simulink model "heli_q8_R_matrix_measurments"  (R2020b)
settings: Solver=ode1  StartTime=0.0  StopTime=inf  FixedStep=0.002  RelTol=1e-3  EnableMultiTasking=on
PostLoadFcn:
  | qc_set_target_type(getConfigSet(bdroot, 'QUARC Default Target Configuration'));
values from neighbouring files (symbols this model uses):
  A_obs = [0 1 0 0 0 ... (first row only)    [init_heli_R_matrix_measurments.m]
  B_obs = [0 0 ... (first row only)    [init_heli_R_matrix_measurments.m]
  C = [1 0 0 0 0 ... (first row only)    [init_heli_R_matrix_measurments.m]
  elevation_offset = 0.5    [init_heli.m]    (also in init_heli_R_matrix_measurments.m)
  F = [K(1,1) K(1,3) ... (first row only)    [init_heli.m]    (also in init_heli_R_matrix_measurments.m)
  Joystick_gain_x = 2    [init_heli.m]    (also in init_heli_R_matrix_measurments.m)
  Joystick_gain_y = -0.5    [init_heli.m]    (also in init_heli_R_matrix_measurments.m)
  K = lqr(A, B, Q, R)    [init_heli.m]    (also in init_heli_R_matrix_measurments.m)
  L = place(A_obs', C', p)'    [init_heli_R_matrix_measurments.m]
undefined symbols (not defined in the file or in its folder): HIL, qc_get_step_size
libraries: quarc_library x9, simulink x4, cstblocks x2, pid_lib x1
settings Model: SimulationMode=external  ExtModeTrigDuration=600000  Creator=Rchan  LastModifiedBy=wiktorjr
settings SolverCC: PositivePriorityOrder=on
settings DataIOCC: LimitDataPoints=on  SaveFormat=Array  SignalLoggingSaveFormat=ModelDataLogs  ReturnWorkspaceOutputs=off
settings OptimizationCC: ExpressionDepthLimit=2147483647  InitFltsAndDblsToZero=on  LifeSpan=inf
settings DebuggingCC: SaveWithParameterizedLinksMsg=none  UnderspecifiedInitializationDetection=Classic  MergeDetectMultiDrivingBlocksExec=none  SolverPrmCheckMsg=warning  MultiTaskDSMMsg=warning  MultiTaskCondExecSysMsg=none  FcnCallInpInsideContextMsg=warning  AllowSymbolicDim=off  StateNameClashWarn=warning  SFUnexpectedBacktrackingDiag=warning  SFNoUnconditionalDefaultTransitionDiag=warning  SFExecutionAtInitializationDiag=none  ArithmeticOperatorsInVariantConditions=warning
settings HardwareCC: ProdBitPerPointer=32  ProdBitPerSizeT=32  ProdBitPerPtrDiffT=32  ProdLargestAtomicFloat=None  ProdIntDivRoundTo=Undefined  ProdEndianess=Unspecified  ProdWordSize=32  ProdHWDeviceType=32-bit Generic
settings ModelReferenceCC: PropagateSignalLabelsOutOfModel=off
settings SFSimCC: SimUseLocalCustomCode=off  CustomCodeUndefinedFunction=UseInterfaceOnly
settings RTWCC: Description=QUARC Win64 Target  SystemTargetFile=quarc_win64.tlc  TemplateMakefile=quarc_default_tmf  RTWUseLocalCustomCode=off
settings CodeAppCC: StateflowObjectComments=on
settings GRTTargetCC: TargetLangStandard=C89/C90 (ANSI)  ParMdlRefBuildCompliant=off  CompOptLevelCompliant=off  CombineOutputUpdateFcns=off  MatFileLogging=off  GRTInterface=on  UseToolchainInfoCompliant=off  ExtMode=on  ExtModeMexFile=quarc_comm
settings ConfigComp: CovMetricSettings=dw  CovSaveCumulativeToWorkspaceVar=on  CovSaveSingleToWorkspaceVar=on  CovExternalEMLEnable=off  CovSFcnEnable=off

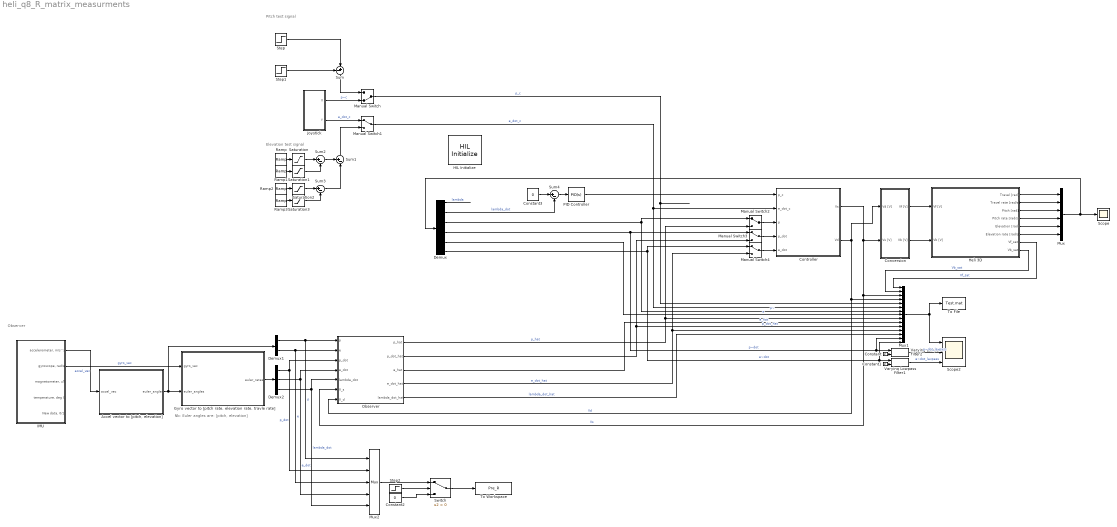
== system heli_q8_R_matrix_measurments ==
  note: Observer
  note: Pitch test signal
  note: Elevation test signal
  note: Nb: Euler angles are: [pitch, elevation]
  "Accel vector to [pitch, elevation]" : MATLAB Function  TreatAsAtomicUnit=on
  Constant : Constant  Value=2
  Constant1 : Constant  Value=2
  Constant2 : Constant  Value=0
  Constant3 : Constant  Value=0
  Controller : Subsystem
  Conversion : Subsystem
  Demux : Demux  Outputs=6
  Demux1 : Demux  Outputs=2
  Demux2 : Demux  Outputs=3
  "Gyro vector to [pitch rate, elevation rate, travle rate]" : MATLAB Function  TreatAsAtomicUnit=on
  HIL Initialize : quarc_library/Data Acquisition/Generic/Configuration/HIL Initialize  Priority=-99  object_name=HIL-1  board_type=q8_usb  board_number=0  board_options=update_rate=normal;decimation=1  exclusive=off  active=off  hardware_clocks=[0:2]  clock_modes=[]  initial_clock_frequencies=[]  set_clock_params_at_start=off  set_clock_params_at_switch_in=off  set_clock_frequencies_at_start=off  set_clock_frequencies_at_switch_in=off  analog_input_channels=[0:7]  analog_input_configurations=[]  analog_input_maximums=10  analog_input_minimums=-10  set_analog_input_params_at_start=on  set_analog_input_params_at_switch_in=off  analog_output_channels=[0:7]  analog_output_maximums=10  analog_output_minimums=-10  initial_analog_outputs=[0]  final_analog_outputs=[0]  watchdog_analog_outputs=0  set_analog_output_params_at_start=on  set_analog_output_params_at_switch_in=off  set_analog_outputs_at_start=on  set_analog_outputs_at_switch_in=off  set_analog_outputs_at_terminate=on  set_analog_outputs_at_switch_out=off  set_analog_outputs_on_watchdog=off  digital_input_channels=[]  digital_output_channels=[]  digital_output_configuration=[]  initial_digital_outputs=[1]  final_digital_outputs=[1]  watchdog_digital_outputs=[1]  set_digital_output_params_at_start=off  set_digital_output_params_at_switch_in=off  set_digital_outputs_at_start=on  set_digital_outputs_at_switch_in=off  set_digital_outputs_at_terminate=on  set_digital_outputs_at_switch_out=off  set_digital_outputs_on_watchdog=off  encoder_channels=[0:7]  quadrature=[4]  encoder_filter_frequency=[]  initial_encoder_counts=[0]  set_encoder_params_at_start=on  set_encoder_params_at_switch_in=off  set_encoder_counts_at_start=on  set_encoder_counts_at_switch_in=off  pwm_channels=[0:7]  pwm_modes=0  pwm_frequency=99.532799999999995e6/4095  pwm_configuration=[0]  pwm_alignment=[0]  pwm_polarity=[1]  pwm_leading_deadband=[0]  pwm_trailing_deadband=[0]  initial_pwm_outputs=[0]  final_pwm_outputs=[0]  watchdog_pwm_outputs=[0]  set_pwm_params_at_start=on  set_pwm_params_at_switch_in=off  set_pwm_outputs_at_start=on  set_pwm_outputs_at_switch_in=off  set_pwm_outputs_at_terminate=on  set_pwm_outputs_at_switch_out=off  set_pwm_outputs_on_watchdog=off  other_output_channels=[]  initial_other_outputs=[]  final_other_outputs=[]  watchdog_other_outputs=[]  set_other_outputs_at_start=off  set_other_outputs_at_switch_in=off  set_other_outputs_at_terminate=off  set_other_outputs_at_switch_out=off  set_other_outputs_on_watchdog=off
  Heli 3D : Subsystem
  IMU : Subsystem
  Joystick : Subsystem
  Manual Switch : ManualSwitch  CurrentSetting=0
  Manual Switch{1..4} (4 alike) : ManualSwitch
  Mux : Mux  Inputs=6
  Mux1 : Mux  Inputs=15
  Mux2 : Mux  Inputs=5
  Observer : Subsystem
  PID Controller : pid_lib/PID Controller  Controller=PID  Form=Parallel  TimeDomain=Continuous-time  UseExternalTs=off  SampleTime=-1  IntegratorMethod=Forward Euler  FilterMethod=Forward Euler  ControllerParametersSource=internal  P=1  I=0.2  D=0  UseFilter=on  N=100  TunerSelectOption=Transfer Function Based (PID Tuner App)  InitialConditionSource=internal  InitialConditionForIntegrator=0  InitialConditionForFilter=0  DifferentiatorICPrevScaledInput=0  ExternalReset=none  TrackingMode=off  Kt=1  LimitOutput=off  SatLimitsSource=internal  UpperSaturationLimit=inf  LowerSaturationLimit=-inf  LinearizeAsGain=on  AntiWindupMode=none  Kb=1  POutMin=[]  POutMax=[]  IOutMin=[]  IOutMax=[]  DOutMin=[]  DOutMax=[]  NOutMin=[]  NOutMax=[]  SumOutMin=[]  SumOutMax=[]  SaturationOutMin=[]  SaturationOutMax=[]  PParamMin=[]  PParamMax=[]  IParamMin=[]  IParamMax=[]  DParamMin=[]  DParamMax=[]  NParamMin=[]  NParamMax=[]  KbParamMin=[]  KbParamMax=[]  KtParamMin=[]  KtParamMax=[]  KbOutMin=[]  KbOutMax=[]  KtOutMin=[]  KtOutMax=[]  IntegratorOutMin=[]  IntegratorOutMax=[]  FilterOutMin=[]  FilterOutMax=[]  SumI1OutMin=[]  SumI1OutMax=[]  SumI2OutMin=[]  SumI2OutMax=[]  SumI3OutMin=[]  SumI3OutMax=[]  SumI4OutMin=[]  SumI4OutMax=[]  SumDOutMin=[]  SumDOutMax=[]  DifferentiatorOutMin=[]  DifferentiatorOutMax=[]  FilterDiffOutCoefMin=[]  FilterDiffOutCoefMax=[]  ReciprocalOutMin=[]  ReciprocalOutMax=[]  SumDenOutMin=[]  SumDenOutMax=[]  SumNumOutMin=[]  SumNumOutMax=[]  DivideOutMin=[]  DivideOutMax=[]  UdiffTsProdOutMin=[]  UdiffTsProdOutMax=[]  NTsProdOutMin=[]  NTsProdOutMax=[]  UintegralTsProdOutMin=[]  UintegralTsProdOutMax=[]  UngainTsProdOutMin=[]  UngainTsProdOutMax=[]  IntegratorContinuousStateAttributes=''  IntegratorStateMustResolveToSignalObject=off  IntegratorRTWStateStorageClass=Auto  FilterContinuousStateAttributes=''  FilterStateMustResolveToSignalObject=off  FilterRTWStateStorageClass=Auto  ParallelPVariant=InternalParameters  IdealPVariant=Disabled  IVariant=InternalParameters  DVariant=InternalParameters  IntegratorVariant=Continuous  SatVariant=Disabled  AWVariant=Passthrough  PCopyVariant=Disabled  TRVariant=Disabled  FdbkBlocksVariant=Forward  IdealPFdbkVariant=Disabled  SatFdbkVariant=Disabled  DerivativeFilterVariant=ContFilter  NVariant=InternalParameters  NCopyVariant=Disabled  FilterICVariant=InternalICsFilter  IntegratorICVariant=InternalICs  ExternalResetVariant=Disabled  TRSumVariant=Passthrough  SumFdbkVariant=Disabled  SumVariant=Sum_PID  TsampFilterVariant=InternalTs  TsampNgainVariant=Passthrough  TsampIntegralVariant=Passthrough  ExternalSaturationOutDataTypeStr=Inherit: Same as second input
  Ramp : simulink/Sources/Ramp  slope=0.03  start=0  InitialOutput=0
  Ramp1 : simulink/Sources/Ramp  slope=0.03  start=4.85  InitialOutput=0
  Ramp2 : simulink/Sources/Ramp  slope=0.03  start=65  InitialOutput=0
  Ramp3 : simulink/Sources/Ramp  slope=0.03  start=70  InitialOutput=0
  Saturation : Saturate  UpperLimit=0.15  LowerLimit=0
  Saturation1 : Saturate  UpperLimit=0.15  LowerLimit=0
  Saturation2 : Saturate  UpperLimit=0.15  LowerLimit=0
  Saturation3 : Saturate  UpperLimit=0.13  LowerLimit=0
  Scope : Scope
  Scope2 : Scope  NumInputPorts=3
  Step : Step  Time=10  After=pi/8  SampleTime=0
  Step1 : Step  Time=40  After=pi/8  SampleTime=0
  Step2 : Step  Time=11  SampleTime=0
  Sum : Sum  Inputs=-+|
  Sum1 : Sum  Inputs=+-|
  Sum2 : Sum  Inputs=|+-
  Sum3 : Sum  Inputs=|+-
  Sum4 : Sum  Inputs=|+-
  Switch : Switch  Criteria=u2 > Threshold
  To File : ToFile  Filename=Test.mat
  To Workspace : ToWorkspace  VariableName=Pre_R  SampleTime=-1
  Varying Lowpass Filter1 : cstblocks/Linear Parameter Varying/Varying Lowpass Filter  N=1
  Varying Lowpass Filter2 : cstblocks/Linear Parameter Varying/Varying Lowpass Filter  N=1
  wires:
  Conversion/2(Vb [V]) -> Heli 3D/2(Vb [V])
  Conversion/1(Vf [V]) -> Heli 3D/1(Vf [V])
  Heli 3D/1(Travel [rad]) -> Mux/1
  Heli 3D/2(Travel rate [rad/s]) -> Mux/2
  Heli 3D/3(Pitch [rad]) -> Mux/3
  Heli 3D/4(Pitch rate [rad/s]) -> Mux/4
  Heli 3D/5(Elevation [rad]) -> Mux/5
  Heli 3D/6(Elevation rate [rad/s]) -> Mux/6
  Mux/1 -> Demux/1, Scope/1
  Mux1/1 -> To File/1, Scope2/1
  Controller/2(Vd) -> Conversion/1(Vd [V]), Observer/7(V_d), Mux1/4  "Vd"
  Demux/3 -> Mux1/7, Manual Switch2/1  "p~"
  Demux/4 -> Mux1/14, Varying Lowpass Filter2/1, Manual Switch3/1  "p~dot"
  Demux/6 -> Mux1/15, Varying Lowpass Filter1/1, Manual Switch4/1  "e~dot"
  Manual Switch/1 -> Mux1/5  "p_c"
  Manual Switch1/1 -> Controller/2(e_dot_c), Mux1/6  "e_dot_c"
  Joystick/2(Y) -> Manual Switch1/1  "e_dot_c"
  Joystick/1(X) -> Manual Switch/2  "p~c"
  Controller/1(Vs) -> Conversion/2(Vs [V]), Observer/6(V_s), Mux1/3  "Vs"
  Constant1/1 -> Varying Lowpass Filter1/2
  Constant/1 -> Varying Lowpass Filter2/2
  Varying Lowpass Filter2/1 -> Scope2/2  "p~dot_lavpass"
  Varying Lowpass Filter1/1 -> Scope2/3  "e~dot_lavpass"
  Sum/1 -> Manual Switch/1
  Step/1 -> Sum/2
  Step1/1 -> Sum/1
  Sum1/1 -> Manual Switch1/2
  Ramp/1 -> Saturation/1
  Saturation/1 -> Sum2/1
  Sum2/1 -> Sum1/1
  Ramp1/1 -> Saturation1/1
  Saturation1/1 -> Sum2/2
  Saturation3/1 -> Sum3/2
  Ramp3/1 -> Saturation3/1
  Saturation2/1 -> Sum3/1
  Ramp2/1 -> Saturation2/1
  Sum3/1 -> Sum1/2
  Heli 3D/8(Vb_sat) -> Mux1/2  "Vb_sat"
  Heli 3D/7(Vf_sat) -> Mux1/1  "Vf_sat"
  IMU/1("accelerometer, m/s^2") -> "Accel vector to [pitch, elevation]"/1(accel_vec)  "accel_vec"
  IMU/2("gyroscope, rad/s") -> "Gyro vector to [pitch rate, elevation rate, travle rate]"/1(gyro_vec)  "gyro_vec"
  "Accel vector to [pitch, elevation]"/1(euler_angles) -> Demux1/1, "Gyro vector to [pitch rate, elevation rate, travle rate]"/2(euler_angles)
  "Gyro vector to [pitch rate, elevation rate, travle rate]"/1(euler_rates) -> Demux2/1
  Demux1/1 -> Mux2/1, Observer/1(p)  "p"
  Demux1/2 -> Mux2/3, Observer/2(e)  "e"
  Demux2/1 -> Mux2/2, Observer/3(p_dot)  "p_dot"
  Demux2/2 -> Observer/4(e_dot), Mux2/4  "e_dot"
  Demux2/3 -> Mux2/5, Observer/5(lambda_dot)  "lambda_dot"
  Observer/1(p_hat) -> Manual Switch2/2, Mux1/9  "p_hat"
  Observer/3(e_hat) -> Mux1/10  "e_hat"
  Observer/2(p_dot_hat) -> Manual Switch3/2, Mux1/11  "p_dot_hat"
  Observer/4(e_dot_hat) -> Manual Switch4/2, Mux1/12  "e_dot_hat"
  Observer/5(lambda_dot_hat) -> Mux1/13  "lambda_dot_hat"
  Demux/5 -> Mux1/8  "e"
  Mux2/1 -> Switch/1
  Switch/1 -> To Workspace/1
  Step2/1 -> Switch/2
  Constant2/1 -> Switch/3
  Demux/2 -> Sum4/2  "lambda_dot"
  Demux/1 -> ?  "lambda"
  Manual Switch2/1 -> Controller/3(p)
  Manual Switch3/1 -> Controller/4(p_dot)
  Manual Switch4/1 -> Controller/5(e_dot)
  PID Controller/1 -> Controller/1(p_c)
  Sum4/1 -> PID Controller/1
  Constant3/1 -> Sum4/1

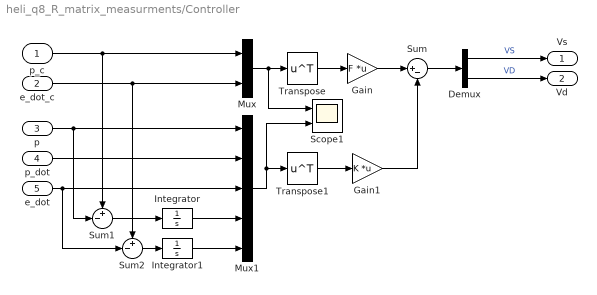
== system heli_q8_R_matrix_measurments/Controller ==
  p_c : Inport
  e_dot_c : Inport  Port=2
  p : Inport  Port=3
  p_dot : Inport  Port=4
  e_dot : Inport  Port=5
  Demux : Demux  Outputs=2
  Gain : Gain  Gain=F  Multiplication=Matrix(K*u) (u vector)
  Gain1 : Gain  Gain=K  Multiplication=Matrix(K*u) (u vector)
  Integrator : Integrator
  Integrator1 : Integrator
  Mux : Mux  Inputs=2
  Mux1 : Mux  Inputs=5
  Scope1 : Scope  NumInputPorts=2
  Sum : Sum  Inputs=|+-
  Sum1 : Sum  Inputs=+-|
  Sum2 : Sum  Inputs=+-|
  Transpose : Math  Operator=transpose  SaturateOnIntegerOverflow=on
  Transpose1 : Math  Operator=transpose  SaturateOnIntegerOverflow=on
  Vs : Outport
  Vd : Outport  Port=2
  wires:
  p_c/1 -> Sum1/1, Mux/1
  p/1 -> Sum1/2, Mux1/1
  p_dot/1 -> Mux1/2
  e_dot/1 -> Sum2/2, Mux1/3
  Mux/1 -> Scope1/1, Transpose/1
  Mux1/1 -> Scope1/2, Transpose1/1
  Gain/1 -> Sum/1
  Gain1/1 -> Sum/2
  Transpose/1 -> Gain/1
  Transpose1/1 -> Gain1/1
  Sum/1 -> Demux/1
  Demux/1 -> Vs/1  "VS"
  e_dot_c/1 -> Mux/2, Sum2/1
  Demux/2 -> Vd/1  "VD"
  Sum1/1 -> Integrator/1
  Sum2/1 -> Integrator1/1
  Integrator/1 -> Mux1/4
  Integrator1/1 -> Mux1/5

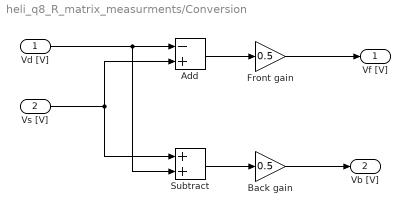
== system heli_q8_R_matrix_measurments/Conversion ==
  Vd [V] : Inport
  Vs [V] : Inport  Port=2
  Add : Sum  Inputs=-+
  Back gain : Gain  Gain=0.5
  Front gain : Gain  Gain=0.5
  Subtract : Sum
  Vf [V] : Outport
  Vb [V] : Outport  Port=2
  wires:
  Vd [V]/1 -> Subtract/2, Add/1
  Vs [V]/1 -> Subtract/1, Add/2
  Subtract/1 -> Back gain/1
  Back gain/1 -> Vb [V]/1
  Add/1 -> Front gain/1
  Front gain/1 -> Vf [V]/1

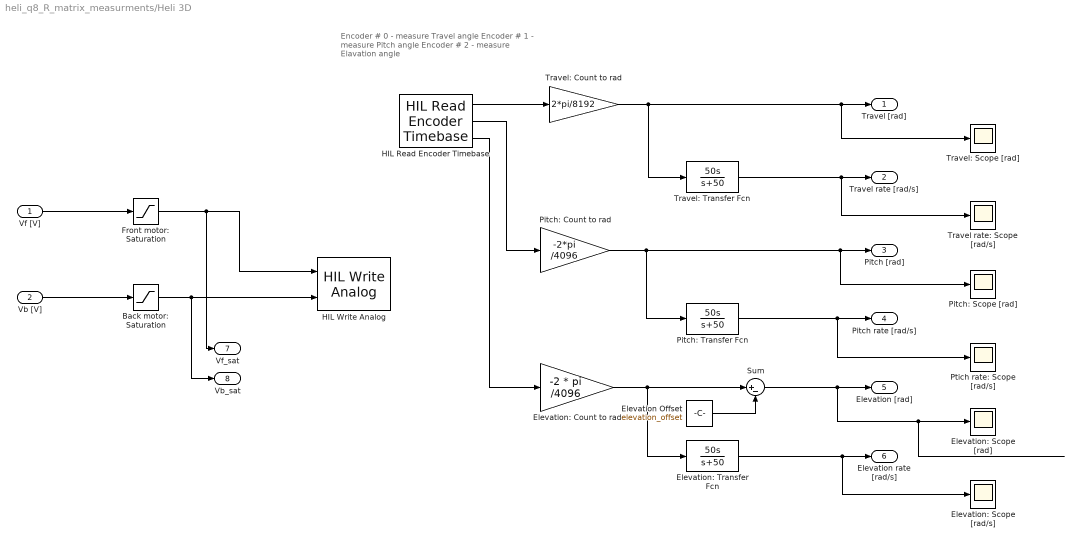
== system heli_q8_R_matrix_measurments/Heli 3D ==
  note: Encoder # 0 - measure Travel angle
      | Encoder # 1 - measure Pitch angle
      | Encoder # 2 - measure Elavation angle
  Vf [V] : Inport
  Vb [V] : Inport  Port=2
  Back motor: Saturation : Saturate  UpperLimit=5  LowerLimit=-5
  Elevation Offset : Constant  Value=elevation_offset
  Elevation: Count to rad : Gain  Gain=-2 * pi /4096
  Elevation: Scope [rad/s] : Scope
  Elevation: Scope [rad] : Scope
  Elevation: Transfer Fcn : TransferFcn  Numerator=[50 0]  Denominator=[1 50]
  Front motor: Saturation : Saturate  UpperLimit=5  LowerLimit=-5
  HIL Read Encoder Timebase : quarc_library/Data Acquisition/Generic/Timebases/HIL Read Encoder Timebase  object_name=HIL-1  clock=0  channels=[0:2]  active=on  vector_output=off  data_type_mode=Inherit via back propagation  data_type=double  overflow_mode=Error on overflow  samples_in_buffer=max(ceil(1/qc_get_step_size), 1)
  HIL Write Analog : quarc_library/Data Acquisition/Generic/Immediate I//O/HIL Write Analog  object_name=HIL-1  channels=[0:1]  sample_time=-1  active=off  vector_input=off
  Pitch: Count to rad : Gain  Gain=-2*pi /4096
  Pitch: Scope [rad] : Scope
  Pitch: Transfer Fcn : TransferFcn  Numerator=[50 0]  Denominator=[1 50]
  Ptich rate: Scope [rad/s] : Scope
  Sum : Sum  Inputs=|+-
  Travel rate: Scope [rad/s] : Scope
  Travel: Count to rad : Gain  Gain=2*pi/8192
  Travel: Scope [rad] : Scope
  Travel: Transfer Fcn : TransferFcn  Numerator=[50 0]  Denominator=[1 50]
  Travel [rad] : Outport
  Travel rate [rad/s] : Outport  Port=2
  Pitch [rad] : Outport  Port=3
  Pitch rate [rad/s] : Outport  Port=4
  Elevation [rad] : Outport  Port=5
  Elevation rate [rad/s] : Outport  Port=6
  Vf_sat : Outport  Port=7
  Vb_sat : Outport  Port=8
  wires:
  HIL Read Encoder Timebase/1 -> Travel: Count to rad/1
  HIL Read Encoder Timebase/2 -> Pitch: Count to rad/1
  HIL Read Encoder Timebase/3 -> Elevation: Count to rad/1
  Travel: Count to rad/1 -> Travel: Scope [rad]/1, Travel [rad]/1, Travel: Transfer Fcn/1
  Travel: Transfer Fcn/1 -> Travel rate: Scope [rad/s]/1, Travel rate [rad/s]/1
  Pitch: Count to rad/1 -> Pitch: Transfer Fcn/1, Pitch: Scope [rad]/1, Pitch [rad]/1
  Pitch: Transfer Fcn/1 -> Ptich rate: Scope [rad/s]/1, Pitch rate [rad/s]/1
  Elevation: Count to rad/1 -> Sum/1, Elevation: Transfer Fcn/1
  Elevation: Transfer Fcn/1 -> Elevation: Scope [rad/s]/1, Elevation rate [rad/s]/1
  Vf [V]/1 -> Front motor: Saturation/1
  Vb [V]/1 -> Back motor: Saturation/1
  Front motor: Saturation/1 -> Vf_sat/1, HIL Write Analog/1
  Back motor: Saturation/1 -> Vb_sat/1, HIL Write Analog/2
  Sum/1 -> Elevation: Scope [rad]/1, Elevation [rad]/1
  Elevation Offset/1 -> Sum/2

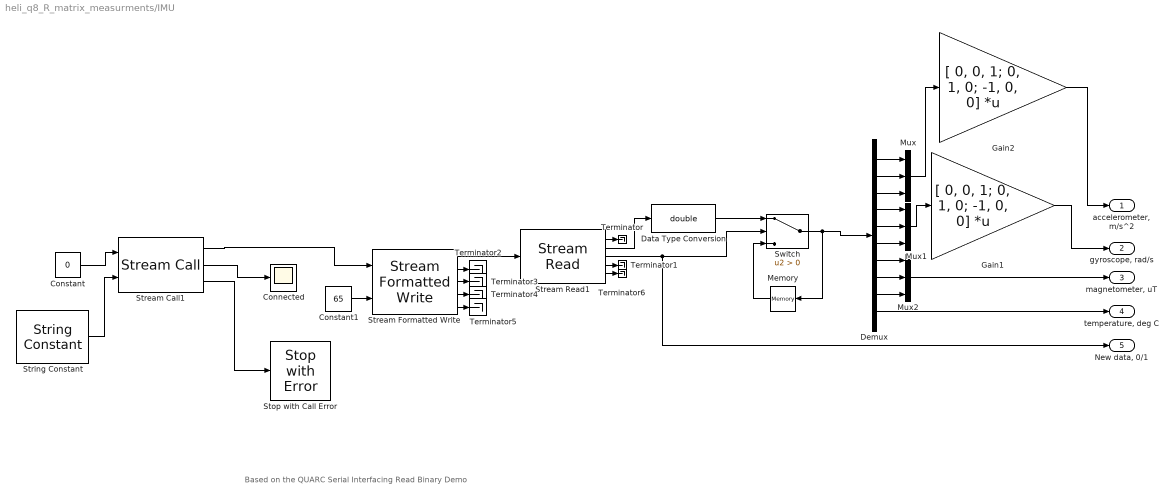
== system heli_q8_R_matrix_measurments/IMU ==
  note: Based on the QUARC Serial Interfacing Read Binary Demo
  Connected : Scope
  Constant : Constant  Value=0
  Constant1 : Constant  Value=65
  Data Type Conversion : DataTypeConversion  OutDataTypeStr=double
  Demux : Demux  Outputs=10
  Gain1 : Gain  Gain=[ 0, 0, 1; 0, 1, 0; -1, 0, 0]  Multiplication=Matrix(K*u) (u vector)
  Gain2 : Gain  Gain=[ 0, 0, 1; 0, 1, 0; -1, 0, 0]  Multiplication=Matrix(K*u) (u vector)
  Memory : Memory  InitialCondition=[0 0 0 0 0 0 0 0 0 0]
  Mux : Mux  Inputs=3
  Mux1 : Mux  Inputs=3
  Mux2 : Mux  Inputs=3
  Stop with Call Error : quarc_library/Sinks/Error Handling/Stop with Error  message_type=Interpret input as error code  message=Error occurred
      settings: SourceProductName=QUARC Targets
  Stream Call1 : quarc_library/Communications/Intermediate/Stream Call  uri_source=External input port  uri=serial://IMU:9?baud=115200,word=8,parity=none,stop=1,flow='none'  apply_uri_to_all_configs=on  send_buffer_size=8000  receive_buffer_size=8000  byte_order=little endian (Intel - LSB first)  sample_time=qc_get_step_size  non_blocking=on  active=off
      settings: SourceProductName=QUARC Targets
  Stream Formatted Write : quarc_library/Communications/Intermediate/Stream Formatted Write  format_string=%c\n  max_code_units=80  optimization=Minimizing latency
      settings: SourceProductName=QUARC Targets
  Stream Read1 : quarc_library/Communications/Intermediate/Stream Read  data_type=single  type_expr=BusObject  num_elements=10  receive_dims=off
      settings: SourceProductName=QUARC Targets
  String Constant : quarc_library/Strings/String Constant  string_value=qc_perform_substitutions('serial://IMU:%{PORT}?baud=115200,word=8,parity=none,stop=1')  evaluate_string=on  string_type=URI  max_length=255  sample_time=inf  variable_size=off
      settings: AttributesFormatString="\"serial://IMU:3?baud=115200,word=8,parity=none,stop=1\""  SourceProductName=QUARC Targets
  Switch : Switch  Criteria=u2 > Threshold
  Terminator{,1..6} (7 alike) : Terminator
  "accelerometer, m/s^2" : Outport
  "gyroscope, rad/s" : Outport  Port=2
  "magnetometer, uT" : Outport  Port=3
  "temperature, deg C" : Outport  Port=4
  "New data, 0/1" : Outport  Port=5
  wires:
  Switch/1 -> Memory/1, Demux/1
  Data Type Conversion/1 -> Switch/1
  Stream Read1/3 -> "New data, 0/1"/1, Switch/2
  Stream Formatted Write/1 -> Stream Read1/1
  Constant1/1 -> Stream Formatted Write/2
  Gain1/1 -> "gyroscope, rad/s"/1
  Gain2/1 -> "accelerometer, m/s^2"/1
  Stream Read1/4 -> Terminator1/1
  Demux/10 -> "temperature, deg C"/1
  Mux1/1 -> Gain1/1
  Stream Read1/2 -> Data Type Conversion/1
  Demux/7 -> Mux2/1
  Demux/8 -> Mux2/2
  Demux/9 -> Mux2/3
  Mux2/1 -> "magnetometer, uT"/1
  Demux/6 -> Mux1/3
  Demux/5 -> Mux1/2
  Demux/4 -> Mux1/1
  Mux/1 -> Gain2/1
  Demux/3 -> Mux/3
  Demux/1 -> Mux/1
  Demux/2 -> Mux/2
  Stream Read1/1 -> Terminator/1
  Stream Call1/1 -> Stream Formatted Write/1
  Constant/1 -> Stream Call1/1
  String Constant/1 -> Stream Call1/2
  Stream Call1/2 -> Connected/1
  Stream Call1/3 -> Stop with Call Error/1
  Memory/1 -> Switch/3
  Stream Formatted Write/2 -> Terminator2/1
  Stream Formatted Write/3 -> Terminator3/1
  Stream Formatted Write/4 -> Terminator4/1
  Stream Formatted Write/5 -> Terminator5/1
  Stream Read1/5 -> Terminator6/1

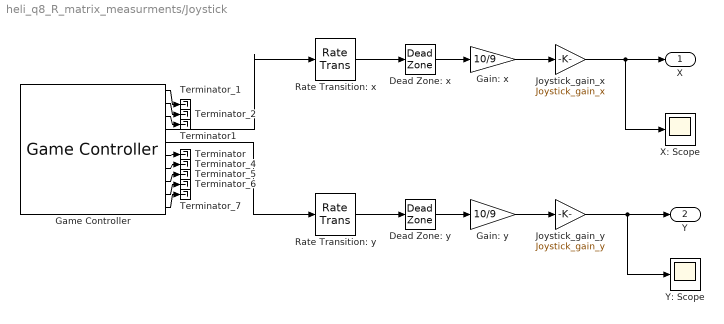
== system heli_q8_R_matrix_measurments/Joystick ==
  Dead Zone: x : DeadZone  LowerValue=-0.1  UpperValue=0.1  SaturateOnIntegerOverflow=on
  Dead Zone: y : DeadZone  LowerValue=-0.1  UpperValue=0.1  SaturateOnIntegerOverflow=on
  Gain: x : Gain  Gain=10/9
  Gain: y : Gain  Gain=10/9
  Game Controller : quarc_library/Devices/Peripherals/Target/Game Controller  controller=1  buffer_size=12  deadzone=[]  saturation=[]  sample_time=max(qc_get_step_size, 0.01)  auto_center=off  enabled=on
      settings: SourceProductName=QUARC Targets
  Joystick_gain_x : Gain  Gain=Joystick_gain_x
  Joystick_gain_y : Gain  Gain=Joystick_gain_y
  Rate Transition: x : RateTransition
  Rate Transition: y : RateTransition
  Terminator : Terminator
  Terminator1 : Terminator
  Terminator_{1..2,4..7} (6 alike) : Terminator
  X: Scope : Scope
  Y: Scope : Scope
  X : Outport
  Y : Outport  Port=2
  wires:
  Rate Transition: y/1 -> Dead Zone: y/1
  Rate Transition: x/1 -> Dead Zone: x/1
  Game Controller/5 -> Rate Transition: y/1
  Game Controller/4 -> Rate Transition: x/1
  Game Controller/1 -> Terminator_1/1
  Game Controller/2 -> Terminator_2/1
  Game Controller/7 -> Terminator_4/1
  Game Controller/8 -> Terminator_5/1
  Game Controller/9 -> Terminator_6/1
  Game Controller/10 -> Terminator_7/1
  Game Controller/3 -> Terminator1/1
  Game Controller/6 -> Terminator/1
  Dead Zone: x/1 -> Gain: x/1
  Dead Zone: y/1 -> Gain: y/1
  Gain: x/1 -> Joystick_gain_x/1
  Gain: y/1 -> Joystick_gain_y/1
  Joystick_gain_x/1 -> X/1, X: Scope/1
  Joystick_gain_y/1 -> Y: Scope/1, Y/1

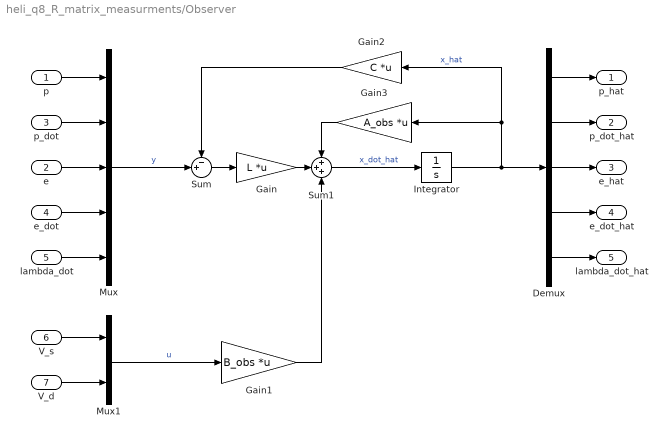
== system heli_q8_R_matrix_measurments/Observer ==
  p : Inport
  e : Inport  Port=2
  p_dot : Inport  Port=3
  e_dot : Inport  Port=4
  lambda_dot : Inport  Port=5
  V_s : Inport  Port=6
  V_d : Inport  Port=7
  Demux : Demux  Outputs=5
  Gain : Gain  Gain=L  Multiplication=Matrix(K*u) (u vector)
  Gain1 : Gain  Gain=B_obs  Multiplication=Matrix(K*u) (u vector)
  Gain2 : Gain  Gain=C  Multiplication=Matrix(K*u) (u vector)
  Gain3 : Gain  Gain=A_obs  Multiplication=Matrix(K*u) (u vector)
  Integrator : Integrator
  Mux : Mux  Inputs=5
  Mux1 : Mux  Inputs=2
  Sum : Sum  Inputs=-+|
  Sum1 : Sum  Inputs=+++
  p_hat : Outport
  p_dot_hat : Outport  Port=2
  e_hat : Outport  Port=3
  e_dot_hat : Outport  Port=4
  lambda_dot_hat : Outport  Port=5
  wires:
  p/1 -> Mux/1
  p_dot/1 -> Mux/2
  e_dot/1 -> Mux/4
  lambda_dot/1 -> Mux/5
  Mux/1 -> Sum/2  "y"
  V_s/1 -> Mux1/1
  V_d/1 -> Mux1/2
  Mux1/1 -> Gain1/1  "u"
  Sum/1 -> Gain/1
  Gain2/1 -> Sum/1
  Gain/1 -> Sum1/2
  Gain3/1 -> Sum1/1
  Sum1/1 -> Integrator/1  "x_dot_hat"
  Gain1/1 -> Sum1/3
  Integrator/1 -> Demux/1, Gain2/1, Gain3/1  "x_hat"
  Demux/1 -> p_hat/1
  Demux/2 -> p_dot_hat/1
  Demux/3 -> e_hat/1
  Demux/4 -> e_dot_hat/1
  Demux/5 -> lambda_dot_hat/1
  e/1 -> Mux/3

== matlab function heli_q8_R_matrix_measurments/Gyro vector to [pitch rate, elevation rate, travle rate] ==
  data: gyro_vec input; euler_rates output; euler_angles input
function euler_rates = gyro_vec_to_euler_rates(gyro_vec,euler_angles)
%#codegen
    pitch_gyro_bias_offset = -0.003;
    elevation_gyro_bias_offset = 0.04;
    travel_gyro_bias_offset = 0.0475;

    phi = euler_angles(1);
    theta = euler_angles(2);
    %psi = euler_angles(3);


    T = [1, sin(phi)*tan(theta), cos(phi)*tan(theta);
         0, cos(phi),            -sin(phi);
         0, sin(phi)/cos(theta), cos(phi)/cos(theta)]; 
     
     euler_rates_pre_offset = T*gyro_vec;
euler_rates = [euler_rates_pre_offset(1) + pitch_gyro_bias_offset, euler_rates_pre_offset(2) + elevation_gyro_bias_offset, euler_rates_pre_offset(3) + travel_gyro_bias_offset];

== matlab function heli_q8_R_matrix_measurments/Accel vector to [pitch, elevation] ==
  data: accel_vec input; euler_angles output
function euler_angles = accel_vec_to_euler(accel_vec)
    pitch_bias_offset = 0.025;
    elevation_bias_offset = 0.0325;

    p = -atan2(accel_vec(2), -accel_vec(3)) + pitch_bias_offset; 
    e = atan2(accel_vec(1), sqrt(accel_vec(2)^2 + accel_vec(3)^2)) + elevation_bias_offset;

euler_angles= [p, e];
